simulink model "Master_Active_Suspension_Simulation_Original"  (R2025b)
settings: Solver=VariableStepAuto  StartTime=0.0  StopTime=10.0  RelTol=1e-3
PreLoadFcn:
  | setup_as;
InitFcn:
  | setup_as;
values from neighbouring files (symbols this model uses):
  A = [ 0,                   1,       0,                      -1 ... (first row only)    [plant_model.m]    (also in setup_as.m)
  B = [ 0,         0 ... (first row only)    [plant_model.m]    (also in setup_as.m)
  C = [ 1, 0, 0, 0 ... (first row only)    [plant_model.m]    (also in setup_as.m)
  D = zeros(6, 2)    [plant_model.m]    (also in setup_as.m)
libraries: simulink x6
settings Model: Creator=HP  LastModifiedBy=Santhosh
settings DebuggingCC: AlgebraicLoopMsg=none
settings RTWCC: GPUComputeCapability=3.5

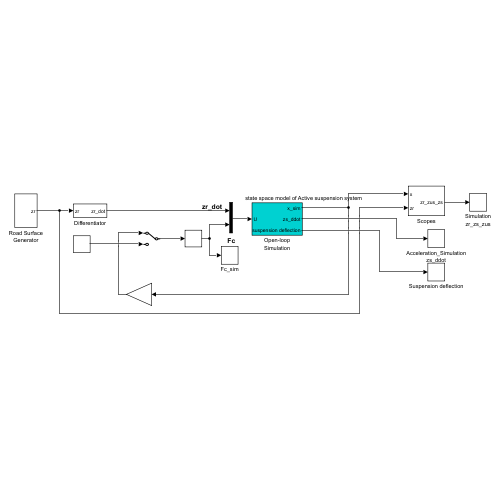
[thumbnail: Simulink's stored preview of the top-level diagram]
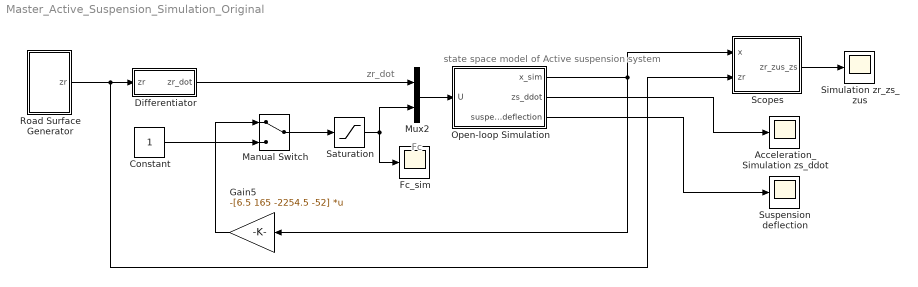
== system Master_Active_Suspension_Simulation_Original ==
  note: state space model of Active suspension system
  note: zr_dot
  note: Fc
  Acceleration_Simulation zs_ddot : Scope
      settings: ActiveDisplayYMinimum=-6.91646  ActiveDisplayYMaximum=6.91642  DataLoggingMaxPoints=300000  DataLoggingVariableName=ScopeData10
  Constant : Constant
  Differentiator : Subsystem
  Fc_sim : Scope
      settings: ActiveDisplayYMinimum=-49  ActiveDisplayYMaximum=49  DataLoggingVariableName=ScopeData3
  Gain5 : Gain  Gain=-[6.5 165 -2254.5 -52]  Multiplication=Matrix(K*u)
  Manual Switch : ManualSwitch
  Mux2 : Mux  Inputs=2
  Open-loop Simulation : Subsystem
  Road Surface Generator : Subsystem
  Saturation : Saturate  UpperLimit=39.2  LowerLimit=-39.2
  Scopes : Subsystem
  Simulation zr_zs_zus : Scope
      settings: ActiveDisplayYMinimum=-0.01485  ActiveDisplayYMaximum=0.03485  DataLoggingMaxPoints=300000
  "Suspension deflection " : Scope
      settings: ActiveDisplayYMinimum=-0.03203  ActiveDisplayYMaximum=0.03201  DataLoggingMaxPoints=300000  DataLoggingVariableName=ScopeData11
  wires:
  Open-loop Simulation/1(x_sim) -> Gain5/1, Scopes/1(x)
  Manual Switch/1 -> Saturation/1
  Scopes/1(zr_zus_zs) -> Simulation zr_zs_zus/1
  Road Surface Generator/1(zr) -> Scopes/2(zr), Differentiator/1(zr)
  Gain5/1 -> Manual Switch/1
  Differentiator/1(zr_dot) -> Mux2/1
  Open-loop Simulation/3(suspension deflection) -> "Suspension deflection "/1
  Saturation/1 -> Mux2/2, Fc_sim/1
  Open-loop Simulation/2(zs_ddot) -> Acceleration_Simulation zs_ddot/1
  Mux2/1 -> Open-loop Simulation/1(U)
  Constant/1 -> Manual Switch/2

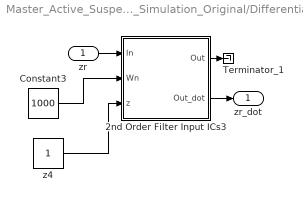
== system Master_Active_Suspension_Simulation_Original/Differentiator ==
  zr : Inport
  2nd Order Filter Input ICs3 : Subsystem
  Constant3 : Constant  Value=1000
  Terminator_1 : Terminator
  z4 : Constant
  zr_dot : Outport  VectorParamsAs1DForOutWhenUnconnected=off
  wires:
  Constant3/1 -> 2nd Order Filter Input ICs3/2(Wn)
  z4/1 -> 2nd Order Filter Input ICs3/3(z)
  zr/1 -> 2nd Order Filter Input ICs3/1(In)
  2nd Order Filter Input ICs3/2(Out_dot) -> zr_dot/1
  2nd Order Filter Input ICs3/1(Out) -> Terminator_1/1

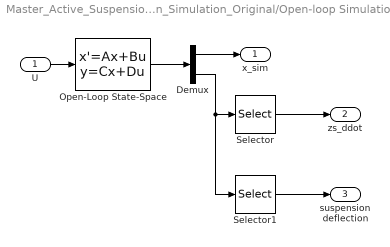
== system Master_Active_Suspension_Simulation_Original/Open-loop Simulation ==
  U : Inport
  Demux : Demux  Outputs=[4 2]
  Open-Loop State-Space : StateSpace  A=A  B=B  C=cat(1,eye(4), C)  D=D  InitialCondition=[0;0;0;0]
  Selector : Selector  InputPortWidth=2  IndexOptions=Index vector (dialog)  Indices=[2]  OutputSizes=1
  Selector1 : Selector  InputPortWidth=2  IndexOptions=Index vector (dialog)  Indices=[1]  OutputSizes=1
  x_sim : Outport  VectorParamsAs1DForOutWhenUnconnected=off
  zs_ddot : Outport  Port=2  VectorParamsAs1DForOutWhenUnconnected=off
  suspension deflection : Outport  Port=3  VectorParamsAs1DForOutWhenUnconnected=off
  wires:
  Open-Loop State-Space/1 -> Demux/1
  Demux/1 -> x_sim/1
  U/1 -> Open-Loop State-Space/1
  Demux/2 -> Selector1/1, Selector/1
  Selector/1 -> zs_ddot/1
  Selector1/1 -> suspension deflection/1

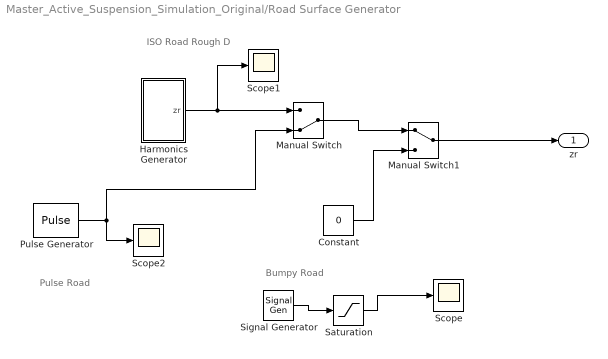
== system Master_Active_Suspension_Simulation_Original/Road Surface Generator ==
  note: Bumpy Road
  note: Pulse Road
  note: ISO Road Rough D
  " Harmonics Generator" : Subsystem
  Constant : Constant  Value=0
  Manual Switch : ManualSwitch  CurrentSetting=0
  Manual Switch1 : ManualSwitch
  Pulse Generator : DiscretePulseGenerator  PulseType=Time based  Amplitude=0.02  Period=4  PulseWidth=50  PhaseDelay=.1
  Saturation : Saturate  UpperLimit=0.02  LowerLimit=0
  Scope : Scope
      settings: ActiveDisplayYMinimum=-0.0025  ActiveDisplayYMaximum=0.0225
  Scope1 : Scope
      settings: ActiveDisplayYMinimum=-0.0025  ActiveDisplayYMaximum=0.0225  DataLoggingVariableName=ScopeData12
  Scope2 : Scope
      settings: ActiveDisplayYMinimum=-0.0025  ActiveDisplayYMaximum=0.0225  DataLoggingVariableName=ScopeData13
  Signal Generator : SignalGenerator  Amplitude=0.02  Frequency=0.2
  zr : Outport  VectorParamsAs1DForOutWhenUnconnected=off
  wires:
  " Harmonics Generator"/1(zr) -> Scope1/1, Manual Switch/1
  Constant/1 -> Manual Switch1/2
  Manual Switch/1 -> Manual Switch1/1
  Manual Switch1/1 -> zr/1
  Signal Generator/1 -> Saturation/1
  Saturation/1 -> Scope/1
  Pulse Generator/1 -> Scope2/1, Manual Switch/2

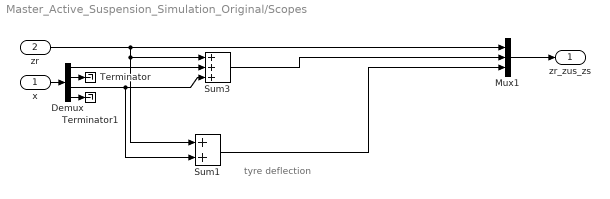
== system Master_Active_Suspension_Simulation_Original/Scopes ==
  note: tyre deflection
  x : Inport
  zr : Inport  Port=2
  Demux : Demux
  Mux1 : Mux  Inputs=3
  Sum1 : Sum  Inputs=2  InputSameDT=on  SaturateOnIntegerOverflow=on  OutDataTypeStr=Inherit: Same as first input
  Sum3 : Sum  Inputs=3  InputSameDT=on  SaturateOnIntegerOverflow=on  OutDataTypeStr=Inherit: Same as first input
  Terminator : Terminator
  Terminator1 : Terminator
  zr_zus_zs : Outport  VectorParamsAs1DForOutWhenUnconnected=off
  wires:
  Demux/1 -> Sum3/2
  Demux/3 -> Sum3/3, Sum1/2
  zr/1 -> Mux1/1, Sum3/1, Sum1/1
  x/1 -> Demux/1
  Mux1/1 -> zr_zus_zs/1
  Demux/2 -> Terminator/1
  Demux/4 -> Terminator1/1
  Sum1/1 -> Mux1/3
  Sum3/1 -> Mux1/2

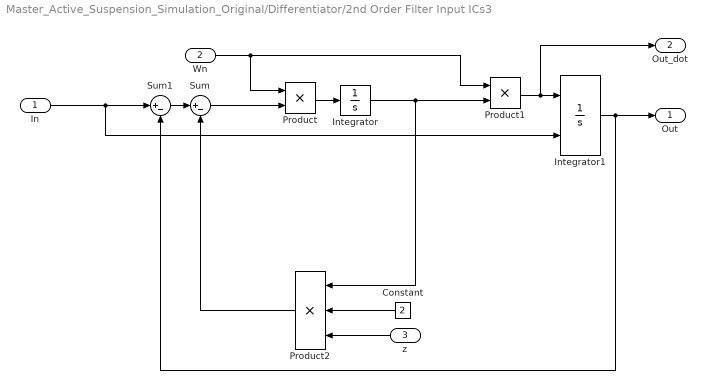
== system Master_Active_Suspension_Simulation_Original/Differentiator/2nd Order Filter Input ICs3 ==
  In : Inport
  Wn : Inport  Port=2
  z : Inport  Port=3
  Constant : Constant  Value=2
  Integrator : Integrator
  Integrator1 : Integrator  InitialConditionSource=external
  Product : Product  RndMeth=Zero
  Product1 : Product  RndMeth=Zero
  Product2 : Product  Inputs=3  RndMeth=Zero
  Sum : Sum  Inputs=|+-
  Sum1 : Sum  Inputs=|+-
  Out : Outport  VectorParamsAs1DForOutWhenUnconnected=off
  Out_dot : Outport  Port=2  VectorParamsAs1DForOutWhenUnconnected=off
  wires:
  Constant/1 -> Product2/2
  z/1 -> Product2/3
  Product2/1 -> Sum/2
  In/1 -> Integrator1/2, Sum1/1
  Sum1/1 -> Sum/1
  Integrator1/1 -> Out/1, Sum1/2
  Integrator/1 -> Product2/1, Product1/2
  Product1/1 -> Out_dot/1, Integrator1/1
  Wn/1 -> Product1/1, Product/1
  Sum/1 -> Product/2
  Product/1 -> Integrator/1

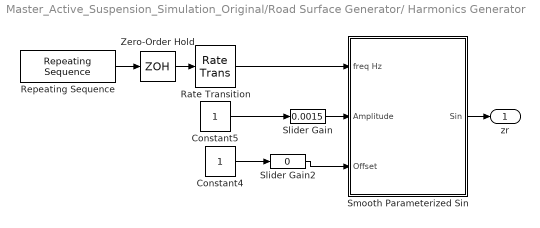
== system Master_Active_Suspension_Simulation_Original/Road Surface Generator/ Harmonics Generator ==
  Constant4 : Constant
  Constant5 : Constant
  Rate Transition : RateTransition
  Repeating Sequence : simulink/Sources/Repeating Sequence  rep_seq_t=[0 30 30.1 ]  rep_seq_y=[1 8 1 ]
  Slider Gain : simulink/Math Operations/Slider Gain  gain=0.0015  low=0  high=0.002
  Slider Gain2 : simulink/Math Operations/Slider Gain  gain=0  low=-10  high=10
  Smooth Parameterized Sin : Subsystem  mask(Smooth Parameterized Sin Wave){}
      mask help:
      | Sin wave that will smoothly and continuously change as input
      | parameters are changed.
      |
      | Out = Amplitude * sin(freq*t) +offset
  Zero-Order Hold : ZeroOrderHold  SampleTime=.1
  zr : Outport  VectorParamsAs1DForOutWhenUnconnected=off
  wires:
  Slider Gain/1 -> Smooth Parameterized Sin/2(Amplitude)
  Slider Gain2/1 -> Smooth Parameterized Sin/3(Offset)
  Constant4/1 -> Slider Gain2/1
  Constant5/1 -> Slider Gain/1
  Repeating Sequence/1 -> Zero-Order Hold/1
  Zero-Order Hold/1 -> Rate Transition/1
  Rate Transition/1 -> Smooth Parameterized Sin/1(freq Hz)
  Smooth Parameterized Sin/1(Sin) -> zr/1

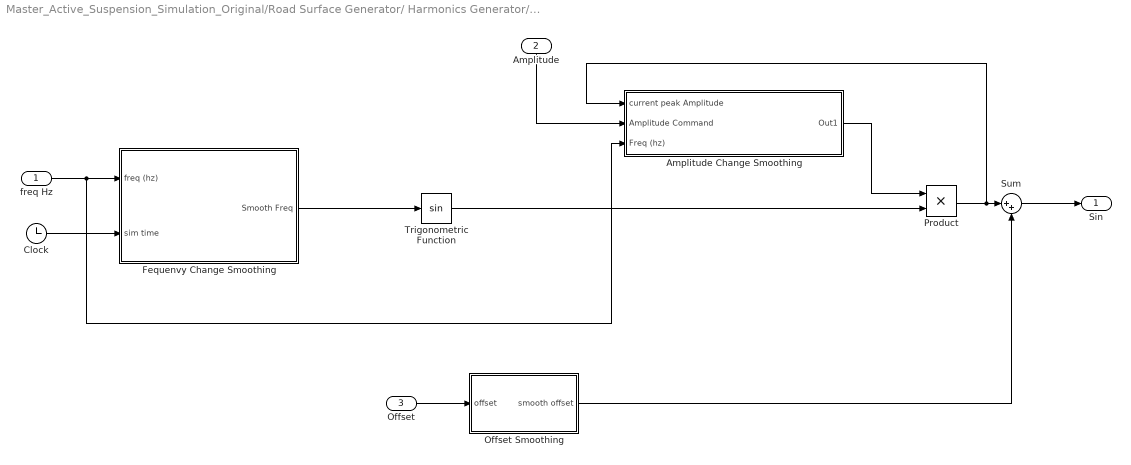
== system Master_Active_Suspension_Simulation_Original/Road Surface Generator/ Harmonics Generator/Smooth Parameterized Sin ==
  freq Hz : Inport
  Amplitude : Inport  Port=2
  Offset : Inport  Port=3
  Amplitude Change Smoothing : Subsystem
  Clock : Clock
  Fequenvy Change Smoothing : Subsystem
  Offset Smoothing : Subsystem
  Product : Product  RndMeth=Zero
  Sum : Sum  Inputs=|++
  Trigonometric Function : Trigonometry
  Sin : Outport  VectorParamsAs1DForOutWhenUnconnected=off
  wires:
  Sum/1 -> Sin/1
  Clock/1 -> Fequenvy Change Smoothing/2(sim time)
  freq Hz/1 -> Fequenvy Change Smoothing/1(freq (hz)), Amplitude Change Smoothing/3(Freq (hz))
  Fequenvy Change Smoothing/1(Smooth Freq) -> Trigonometric Function/1
  Trigonometric Function/1 -> Product/2
  Offset Smoothing/1(smooth offset) -> Sum/2
  Offset/1 -> Offset Smoothing/1(offset)
  Product/1 -> Sum/1, Amplitude Change Smoothing/1(current peak Amplitude)
  Amplitude Change Smoothing/1(Out1) -> Product/1
  Amplitude/1 -> Amplitude Change Smoothing/2(Amplitude Command)

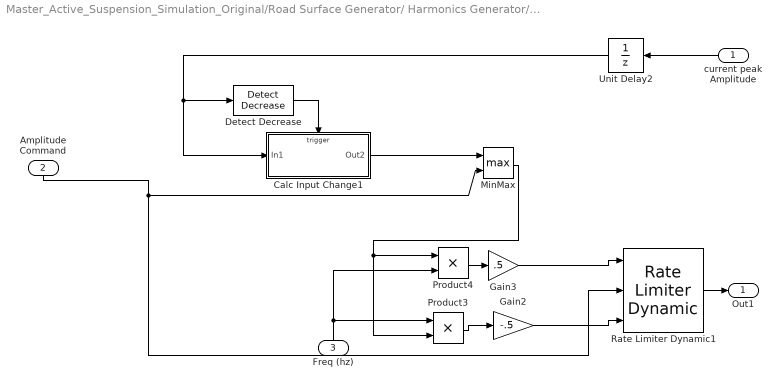
== system Master_Active_Suspension_Simulation_Original/Road Surface Generator/ Harmonics Generator/Smooth Parameterized Sin/Amplitude Change Smoothing ==
  current peak Amplitude : Inport
  Amplitude Command : Inport  Port=2
  Freq (hz) : Inport  Port=3
  Calc Input Change1 : Subsystem  TreatAsAtomicUnit=on
  Detect Decrease : simulink/Logic and Bit Operations/Detect Decrease  vinit=0.0  OutDataTypeStr=uint8
  Gain2 : Gain  Gain=-.5
  Gain3 : Gain  Gain=.5
  MinMax : MinMax  Function=max  Inputs=2
  Product3 : Product  RndMeth=Zero
  Product4 : Product  RndMeth=Zero
  Rate Limiter Dynamic1 : simulink/Discontinuities/Rate Limiter Dynamic
  Unit Delay2 : UnitDelay  SampleTime=-1  HasFrameUpgradeWarning=on
  Out1 : Outport  VectorParamsAs1DForOutWhenUnconnected=off
  wires:
  Gain2/1 -> Rate Limiter Dynamic1/3
  Gain3/1 -> Rate Limiter Dynamic1/1
  Amplitude Command/1 -> MinMax/2, Rate Limiter Dynamic1/2
  Product3/1 -> Gain2/1
  Product4/1 -> Gain3/1
  Detect Decrease/1 -> Calc Input Change1/Trigger
  Calc Input Change1/1(Out2) -> MinMax/1
  Unit Delay2/1 -> Calc Input Change1/1(In1), Detect Decrease/1
  MinMax/1 -> Product4/1, Product3/2
  current peak Amplitude/1 -> Unit Delay2/1
  Freq (hz)/1 -> Product3/1, Product4/2
  Rate Limiter Dynamic1/1 -> Out1/1

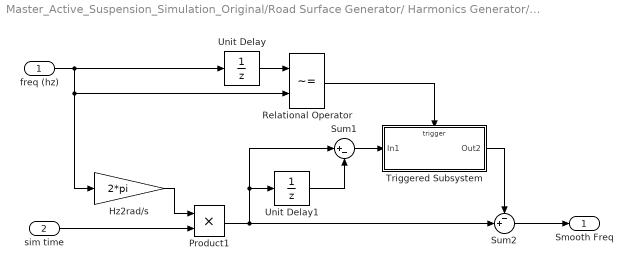
== system Master_Active_Suspension_Simulation_Original/Road Surface Generator/ Harmonics Generator/Smooth Parameterized Sin/Fequenvy Change Smoothing ==
  freq (hz) : Inport
  sim time : Inport  Port=2
  Hz2rad/s : Gain  Gain=2*pi
  Product1 : Product  RndMeth=Zero
  Relational Operator : RelationalOperator  Operator=~=  OutDataTypeStr=boolean  InputSameDT=off
  Sum1 : Sum  Inputs=|+-
  Sum2 : Sum  Inputs=-+|
  Triggered Subsystem : Subsystem  TreatAsAtomicUnit=on
  Unit Delay : UnitDelay  SampleTime=-1  HasFrameUpgradeWarning=on
  Unit Delay1 : UnitDelay  SampleTime=-1  HasFrameUpgradeWarning=on
  Smooth Freq : Outport  VectorParamsAs1DForOutWhenUnconnected=off
  wires:
  Triggered Subsystem/1(Out2) -> Sum2/1
  Unit Delay1/1 -> Sum1/2
  Relational Operator/1 -> Triggered Subsystem/Trigger
  Sum1/1 -> Triggered Subsystem/1(In1)
  Unit Delay/1 -> Relational Operator/1
  Product1/1 -> Sum2/2, Sum1/1, Unit Delay1/1
  freq (hz)/1 -> Unit Delay/1, Relational Operator/2, Hz2rad/s/1
  Sum2/1 -> Smooth Freq/1
  sim time/1 -> Product1/2
  Hz2rad/s/1 -> Product1/1

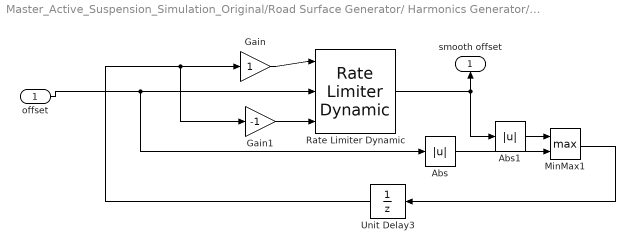
== system Master_Active_Suspension_Simulation_Original/Road Surface Generator/ Harmonics Generator/Smooth Parameterized Sin/Offset Smoothing ==
  offset : Inport
  Abs : Abs  SaturateOnIntegerOverflow=off
  Abs1 : Abs  SaturateOnIntegerOverflow=off
  Gain : Gain
  Gain1 : Gain  Gain=-1
  MinMax1 : MinMax  Function=max  Inputs=2
  Rate Limiter Dynamic : simulink/Discontinuities/Rate Limiter Dynamic
  Unit Delay3 : UnitDelay  SampleTime=-1  HasFrameUpgradeWarning=on
  smooth offset : Outport  VectorParamsAs1DForOutWhenUnconnected=off
  wires:
  Rate Limiter Dynamic/1 -> Abs1/1, smooth offset/1
  offset/1 -> Rate Limiter Dynamic/2, Abs/1
  Gain1/1 -> Rate Limiter Dynamic/3
  Gain/1 -> Rate Limiter Dynamic/1
  MinMax1/1 -> Unit Delay3/1
  Unit Delay3/1 -> Gain/1, Gain1/1
  Abs/1 -> MinMax1/2
  Abs1/1 -> MinMax1/1

== system Master_Active_Suspension_Simulation_Original/Road Surface Generator/ Harmonics Generator/Smooth Parameterized Sin/Amplitude Change Smoothing/Calc Input Change1 ==
  In1 : Inport
  Trigger : TriggerPort  VariantControl=(inherit)
  Out2 : Outport  InitialOutput=1000  VectorParamsAs1DForOutWhenUnconnected=off
  wires:
  In1/1 -> Out2/1

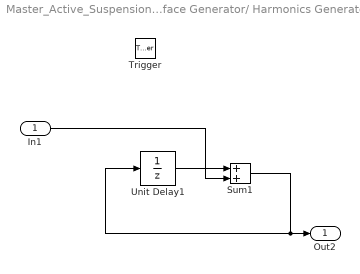
== system Master_Active_Suspension_Simulation_Original/Road Surface Generator/ Harmonics Generator/Smooth Parameterized Sin/Fequenvy Change Smoothing/Triggered Subsystem ==
  In1 : Inport
  Trigger : TriggerPort  VariantControl=(inherit)
  Sum1 : Sum
  Unit Delay1 : UnitDelay  SampleTime=-1  HasFrameUpgradeWarning=on
  Out2 : Outport  InitialOutput=0  VectorParamsAs1DForOutWhenUnconnected=off
  wires:
  Unit Delay1/1 -> Sum1/1
  Sum1/1 -> Unit Delay1/1, Out2/1
  In1/1 -> Sum1/2
